simulink model "bins_model_with_aerospace"  (Simulink 7.9)
settings: Solver=ode45  StartTime=0.0  StopTime=20.0  RelTol=1e-3
libraries: aerolib6dof2 x1, aerolibnav x1
settings Model: Creator=S  LastModifiedBy=S

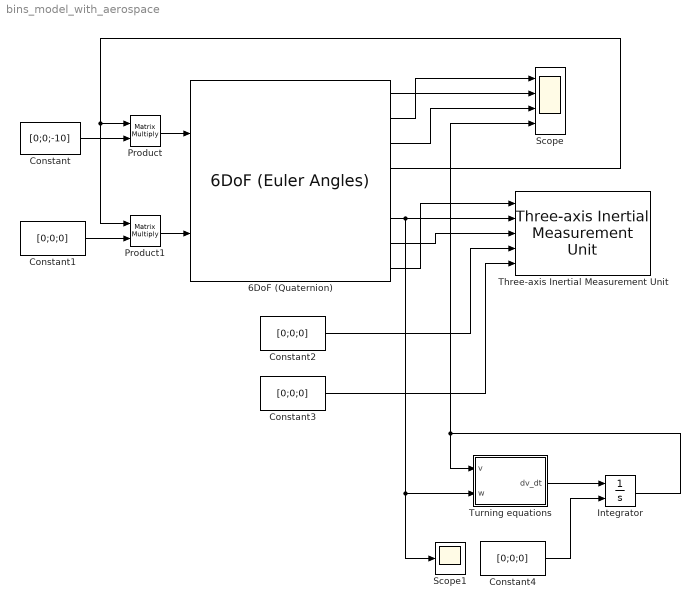
== system bins_model_with_aerospace ==
  6DoF (Quaternion) : aerolib6dof2/6DoF (Euler Angles)  units=Metric (MKS)  mtype=Fixed  rep=Euler Angles  xme_0=[0 0 0]  Vm_0=[100 0 100]  eul_0=[0 0 0]  pm_0=[3 5 2]  mass_0=1.0  mass_e=0  mass_f=0  inertia=eye(3)  inertia_e=eye(3)  inertia_f=eye(3)  k_quat=1.0
  Constant : Constant  Value=[0;0;-10]
  Constant{1..4} (4 alike) : Constant  Value=[0;0;0]
  Integrator : Integrator  InitialConditionSource=external
  Product : Product  Multiplication=Matrix(*)  RndMeth=Zero
  Product1 : Product  Multiplication=Matrix(*)  RndMeth=Zero
  Scope : Scope  NumInputPorts=4
      settings: TimeRange=20  YMin=-1000~-200~0~0  YMax=2000~100~20~20  MaxDataPoints=50000
  Scope1 : Scope
  Three-axis Inertial Measurement Unit : aerolibnav/Three-axis Inertial Measurement Unit  units=Metric (MKS)  imu=[0 0 0]  dtype_a=on  w_a=190  z_a=0.707  a_sf_cc=[1 0 0; 0 1 0; 0 0 1]  a_bias=[0 0 0]  a_sat="[-inf  -inf  -inf  inf inf inf]"  dtype_g=on  w_g=190  z_g=0.707  g_sf_cc=[1 0 0; 0 1 0; 0 0 1]  g_bias=[0 0 0]  g_sens=[0 0 0]  g_sat="[-inf  -inf  -inf  inf inf inf]"  i_rand=on  i_seeds=[23093 23094 23095 23096 23097 23098]  i_pow=[0.001 0.001 0.001 0.0001 0.0001 0.0001]  i_Ts=0
  Turning equations : MATLAB Function  TreatAsAtomicUnit=on
  wires:
  6DoF (Quaternion)/8 -> Three-axis Inertial Measurement Unit/1
  6DoF (Quaternion)/6 -> Three-axis Inertial Measurement Unit/2, Turning equations/2(w), Scope1/1
  6DoF (Quaternion)/7 -> Three-axis Inertial Measurement Unit/3
  Constant/1 -> Product/2
  Constant1/1 -> Product1/2
  Constant2/1 -> Three-axis Inertial Measurement Unit/4
  Constant3/1 -> Three-axis Inertial Measurement Unit/5
  6DoF (Quaternion)/2 -> Scope/1
  6DoF (Quaternion)/1 -> Scope/2
  6DoF (Quaternion)/3 -> Scope/3
  Product/1 -> 6DoF (Quaternion)/1
  Product1/1 -> 6DoF (Quaternion)/2
  6DoF (Quaternion)/4 -> Product/1, Product1/1
  Turning equations/1(dv_dt) -> Integrator/1
  Constant4/1 -> Integrator/2
  Integrator/1 -> Turning equations/1(v), Scope/4

== matlab function Turning equations ==
  data: v input double; dv_dt output double; w input double
function dv_dt = fcn(v, w)
%#codegen

    dv_dt = f_turning_by_Euler2(v, w);
    
end
